simulink model "glassTemp"  (R2025a)
settings: Solver=VariableStepAuto  StartTime=0.0  StopTime=3000.0  RelTol=1e-3
settings Model: Creator=Laurenpearse  LastModifiedBy=Laurenpearse

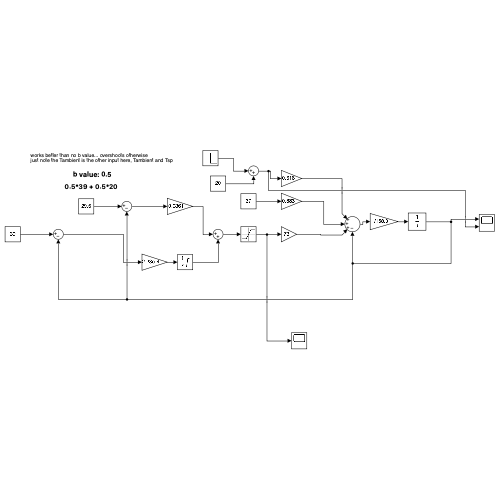
[thumbnail: Simulink's stored preview of the top-level diagram]
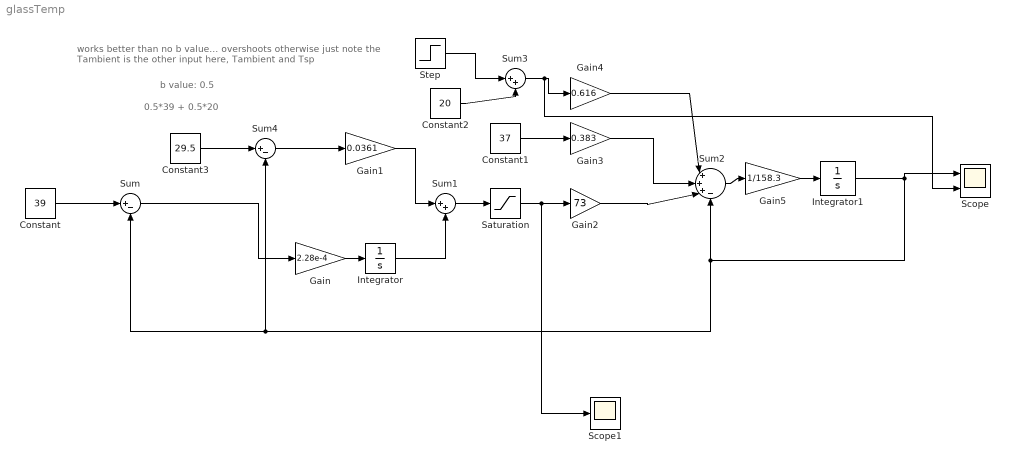
== system glassTemp ==
  note: works better than no b value... overshoots otherwise
      | just note the Tambient is the other input here, Tambient and Tsp
  note: b value: 0.5
  note: 0.5*39 + 0.5*20
  Constant : Constant  Value=39
  Constant1 : Constant  Value=37
  Constant2 : Constant  Value=20
  Constant3 : Constant  Value=29.5
  Gain : Gain  Gain=2.28e-4
  Gain1 : Gain  Gain=0.0361
  Gain2 : Gain  Gain=73
  Gain3 : Gain  Gain=0.383
  Gain4 : Gain  Gain=0.616
  Gain5 : Gain  Gain=1/158.3
  Integrator : Integrator  LimitOutput=on  UpperSaturationLimit=1  LowerSaturationLimit=0
  Integrator1 : Integrator  InitialCondition=20
  Saturation : Saturate  UpperLimit=1  LowerLimit=0
  Scope : Scope  NumInputPorts=2
      settings: ActiveDisplayYMinimum=9.816346668586597  ActiveDisplayYMaximum=46.93494470756383
  Scope1 : Scope
      settings: ActiveDisplayYMinimum=0.14990679206920446  ActiveDisplayYMaximum=0.36439924532564394
  Step : Step  Time=2500  After=-4  SampleTime=0
  Sum : Sum  Inputs=|+-
  Sum1 : Sum  Inputs=|++
  Sum2 : Sum  Inputs=|+++-
  Sum3 : Sum  Inputs=|++
  Sum4 : Sum  Inputs=|+-
  wires:
  Sum3/1 -> Scope/2, Gain4/1
  Sum2/1 -> Gain5/1
  Constant2/1 -> Sum3/2
  Gain3/1 -> Sum2/2
  Gain1/1 -> Sum1/1
  Gain4/1 -> Sum2/1
  Constant/1 -> Sum/1
  Constant1/1 -> Gain3/1
  Integrator/1 -> Sum1/2
  Step/1 -> Sum3/1
  Gain2/1 -> Sum2/3
  Gain5/1 -> Integrator1/1
  Saturation/1 -> Scope1/1, Gain2/1
  Sum1/1 -> Saturation/1
  Integrator1/1 -> Sum2/4, Sum4/2, Sum/2, Scope/1
  Sum/1 -> Gain/1
  Gain/1 -> Integrator/1
  Constant3/1 -> Sum4/1
  Sum4/1 -> Gain1/1
